simulink model "Mega_BalanceCode_r"  (R2023a)
settings: Solver=FixedStepDiscrete  StartTime=0.0  StopTime=inf  FixedStep=TS  RelTol=1e-3  EnableMultiTasking=on
values from neighbouring files (symbols this model uses):
  ES = -C2DEG*D2R    (= -0.00872664625997)    [NXT_Parameters.m]
  GS = GyroS*D2R    (= 0.000155832968928)    [NXT_Parameters.m]
  Ki = 1*[-Rw -Rw*0 1 1*0]    [NXT_Parameters.m]
  KLQRC = KLQR.*[-Rw -Rw 1 1]    [NXT_Parameters.m]
  TS = .005    (= 0.005)    [NXT_Parameters.m]
  tstart = TS*110    (= 0.55)    [NXT_Parameters.m]
  V2DCB = 1/DCB2V    (= 28.3333333333)    [NXT_Parameters.m]
undefined symbols (not defined in the file or in its folder): DiscIntNeverNeededParam
libraries: simulink x2, arduinolib x2
settings Model: FPTRunName=FPA_Reference  SimulationMode=external  ExtModeTrigDuration=2  Creator=Alec  LastModifiedBy=ASUS
settings SolverCC: AlgebraicLoopSolver=TrustRegion
settings DataIOCC: LimitDataPoints=on  SaveFormat=Array  ReturnWorkspaceOutputs=off
settings OptimizationCC: EnhancedBackFolding=on  PassReuseOutputArgsAs=Individual arguments  ExpressionDepthLimit=2147483647  ZeroExternalMemoryAtStartup=off  ZeroInternalMemoryAtStartup=off  MaxStackSize=64  OptimizeBlockOrder=speed  DifferentSizesBufferReuse=on  OptimizationCustomize=off  EfficientTunableParamExpr=on
settings DebuggingCC: UnderspecifiedInitializationDetection=Classic  MergeDetectMultiDrivingBlocksExec=none  ParameterTunabilityLossMsg=error  UnconnectedInputMsg=warning  UnconnectedOutputMsg=warning  UnconnectedLineMsg=warning  StateNameClashWarn=warning  SFUnexpectedBacktrackingDiag=warning  SFNoUnconditionalDefaultTransitionDiag=warning  SFExecutionAtInitializationDiag=none  ArithmeticOperatorsInVariantConditions=warning
settings HardwareCC: ProdBitPerInt=16  ProdBitPerPointer=16  ProdBitPerSizeT=16  ProdBitPerPtrDiffT=16  ProdLargestAtomicFloat=None  ProdWordSize=8  ProdHWDeviceType=Atmel->AVR
settings ModelReferenceCC: PropagateSignalLabelsOutOfModel=off
settings SFSimCC: SimUseLocalCustomCode=off  MATLABDynamicMemAlloc=off  CustomCodeUndefinedFunction=UseInterfaceOnly
settings RTWCC: Description=Embedded Coder  SystemTargetFile=ert.tlc  HardwareBoard=Arduino Mega 2560  TemplateMakefile=ert_default_tmf  RTWVerbose=off  RTWUseLocalCustomCode=off  Toolchain=Arduino AVR  BuildConfiguration=Faster Runs
settings CodeAppCC: ForceParamTrailComments=on  IgnoreCustomStorageClasses=off  OperatorAnnotations=on  SimulinkDataObjDesc=on  SFDataObjDesc=on  CustomSymbolStrType=$N$R$M  InsertBlockDesc=on  InternalIdentifier=Classic
settings ERTTargetCC: SupportContinuousTime=on  SupportVariableSizeSignals=on  ExtModeTransport=3  ExtModeStaticAlloc=on  ExtModeAutomaticAllocSize=off  ExtModeStaticAllocSize=2048  ExtModeMexFile=ext_xcp  ExtModeIntrfLevel=Level2 - Open
settings ConfigComp: CovMetricSettings=dw  CovSaveCumulativeToWorkspaceVar=on  CovSaveSingleToWorkspaceVar=on  CovExternalEMLEnable=off

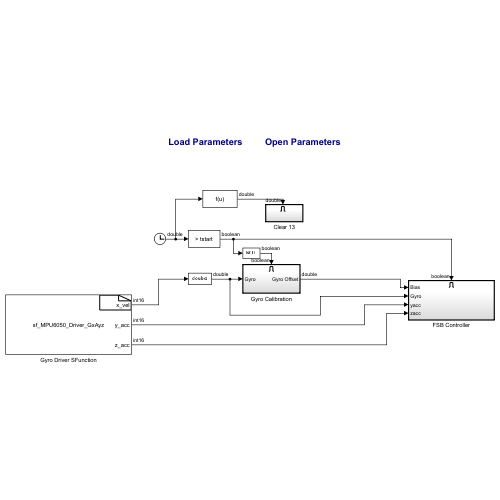
[thumbnail: Simulink's stored preview of the top-level diagram]
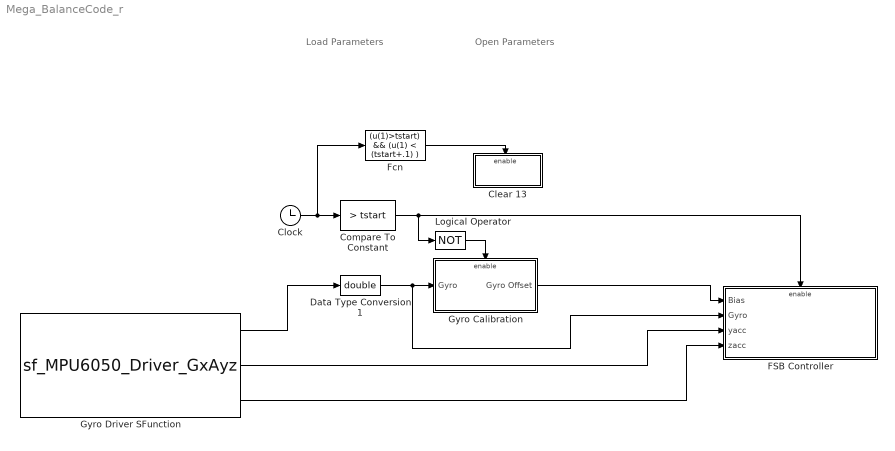
== system Mega_BalanceCode_r ==
  note: Load Parameters
  note: Open Parameters
  "Clear 13 " : Subsystem  TreatAsAtomicUnit=on
  Clock : Clock
  Compare To Constant : simulink/Logic and Bit Operations/Compare To Constant  relop=>  const=tstart  OutDataTypeStr=boolean
  Data Type Conversion1 : DataTypeConversion  OutDataTypeStr=double  SaturateOnIntegerOverflow=off  RndMeth=Floor
  FSB Controller : Subsystem
  Fcn : Fcn  Expr=(u(1)>tstart) && (u(1) < (tstart+.1) )
  Gyro Calibration : Subsystem  TreatAsAtomicUnit=on
  Gyro Driver SFunction : S-Function  InitFcn=try, set_param(gcb,'FunctionName','sf_MPU6050_Driver_GxAyz'), end  FunctionName=sf_MPU6050_Driver_GxAyz  SFunctionModules=sf_MPU6050_Driver_GxAyz_wrapper.cpp  SFunctionDeploymentMode=off  EnableBusSupport=off  mask(S-Function Builder){}
      mask help: Simulink:masks:SFunctionBuilder_MD
      mask init:
      | val = [[.9  0.75 0.75 1 1 .9 .9 1]',[1 1 0.75 0.75 .9 .9 1 .9]'];try , sys = get_param(gcb,'SfunBuilderFcnName');if isempty(sys), sys = get_param(gcb,'FunctionName'); end,catch, sys = get_param(gcb,'FunctionName'); end
      settings: CopyFcn=set_param(gcbh,'LinkStatus','none')  PreSaveFcn=try, set_param(gcb,'FunctionName','sf_MPU6050_Driver_GxAyz'), end  OpenFcn=sfunctionwizard(gcbh)
      mask Display:
      | plot(val(:,1),val(:,2))
      | disp(sys)
      | port_label('output',1,'x_vel')
      | port_label('output',2,'y_acc')
      | port_label('output',3,'z_acc')
  Logical Operator : Logic  Operator=NOT  AllPortsSameDT=off  OutDataTypeStr=boolean
  wires:
  Clock/1 -> Fcn/1, Compare To Constant/1
  Compare To Constant/1 -> Logical Operator/1, FSB Controller/Enable
  Gyro Calibration/1(Gyro Offset) -> FSB Controller/1(Bias)
  Gyro Driver SFunction/1 -> Data Type Conversion1/1
  Logical Operator/1 -> Gyro Calibration/Enable
  Data Type Conversion1/1 -> FSB Controller/2(Gyro), Gyro Calibration/1(Gyro)
  Fcn/1 -> "Clear 13 "/Enable
  Gyro Driver SFunction/2 -> FSB Controller/3("yacc ")
  Gyro Driver SFunction/3 -> FSB Controller/4("zacc ")

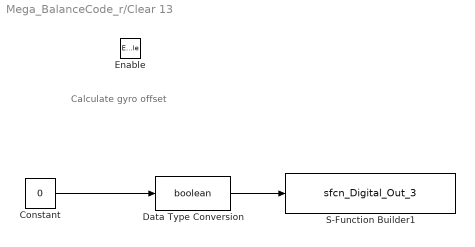
== system Mega_BalanceCode_r/Clear 13  ==
  note: Calculate gyro offset
  Enable : EnablePort
  Constant : Constant  Value=0
  Data Type Conversion : DataTypeConversion  OutDataTypeStr=boolean  SaturateOnIntegerOverflow=off  RndMeth=Floor
  S-Function Builder1 : S-Function  InitFcn=try, set_param(gcb,'FunctionName','sfcn_Digital_Out_3'), end  FunctionName=sfcn_Digital_Out_3  Parameters=uint8(13)  SFunctionModules=sfcn_Digital_Out_3_wrapper  SFunctionDeploymentMode=off  EnableBusSupport=off  mask(S-Function Builder){}
      mask init: same as Mega_BalanceCode_r/Gyro Driver SFunction
      settings: CopyFcn=set_param(gcbh,'LinkStatus','none')  PreSaveFcn=try, set_param(gcb,'FunctionName','sfcn_Digital_Out_3'), end  OpenFcn=sfunctionwizard(gcbh)
      mask Display: plot(val(:,1),val(:,2)),disp(sys), port_label('input',1,'in')
  wires:
  Constant/1 -> Data Type Conversion/1
  Data Type Conversion/1 -> S-Function Builder1/1

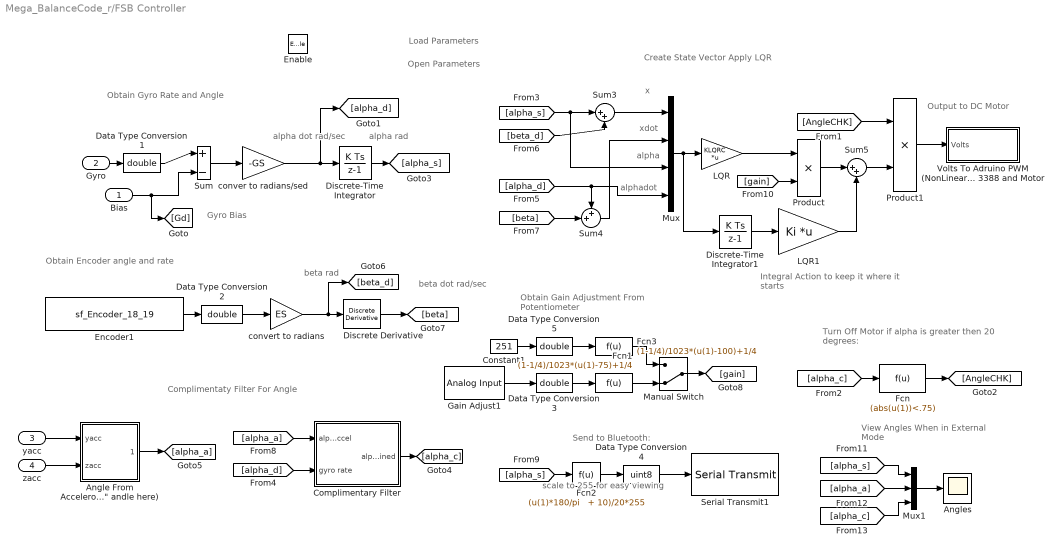
== system Mega_BalanceCode_r/FSB Controller ==
  note: scale to 255 for easy viewing
  note: Integral Action to keep
      |  it where it starts
  note: Gyro
      | Bias
  note: Turn Off Motor if alpha
      | is greater then 20 degrees:
  note: Output to DC Motor
  note: Create State Vector
      | Apply LQR
  note: Obtain Encoder angle
      | and rate
  note: Obtain Gyro Rate
      | and Angle
  note: xdot
  note: x
  note: beta
      | rad
  note: alpha dot
      | rad/sec
  note: alpha
      | rad
  note: beta dot
      | rad/sec
  note: alpha
  note: alphadot
  note: Load Parameters
  note: Open Parameters
  note: Complimentaty Filter
      | For Angle
  note: Obtain Gain Adjustment
      | From Potentiometer
  note: Send to Bluetooth:
  note: View Angles When in
      | External Mode
  Bias : Inport
  Gyro : Inport  Port=2
  "yacc " : Inport  Port=3
  "zacc " : Inport  Port=4
  Enable : EnablePort
  " Complimentary Filter" : Subsystem
  "Angle From Accelerometer (adjust \"zero\" andle here)" : Subsystem
  Angles : Scope
  Constant1 : Constant  Value=251
  Data Type Conversion{1..3,5} (4 alike) : DataTypeConversion  OutDataTypeStr=double  SaturateOnIntegerOverflow=off  RndMeth=Floor
  Data Type Conversion4 : DataTypeConversion  OutDataTypeStr=uint8  SaturateOnIntegerOverflow=off  RndMeth=Floor
  Discrete Derivative : simulink/Discrete/Discrete Derivative  gainval=1.0  ICPrevScaledInput=0.0  OutMin=[]  OutMax=[]  OutDataType=fixdt(1, 16)  OutScaling=2^-10  DoSatur=off
  Discrete-Time Integrator : DiscreteIntegrator  SampleTime=TS  ICPrevOutput=DiscIntNeverNeededParam  ICPrevScaledInput=DiscIntNeverNeededParam
  Discrete-Time Integrator1 : DiscreteIntegrator  SampleTime=TS  ICPrevOutput=DiscIntNeverNeededParam  ICPrevScaledInput=DiscIntNeverNeededParam
  Encoder1 : S-Function  InitFcn=try, set_param(gcb,'FunctionName','sf_Encoder_18_19'), end  FunctionName=sf_Encoder_18_19  Parameters=uint8(0),uint8(18),uint8(19)  SFunctionModules=sf_Encoder_18_19_wrapper  SFunctionDeploymentMode=off  EnableBusSupport=off  mask(S-Function Builder){}
      mask init: same as Mega_BalanceCode_r/Gyro Driver SFunction
      settings: CopyFcn=set_param(gcbh,'LinkStatus','none')  PreSaveFcn=try, set_param(gcb,'FunctionName','sf_Encoder_18_19'), end  OpenFcn=sfunctionwizard(gcbh)
      mask Display: plot(val(:,1),val(:,2)),disp(sys), port_label('output',1,'pos')
  Fcn : Fcn  Expr=(abs(u(1))<.75)
  Fcn1 : Fcn  Expr=(1-1/4)/1023*(u(1)-75)+1/4
  Fcn2 : Fcn  Expr="(u(1)*180/pi   + 10)/20*255"
  Fcn3 : Fcn  Expr=(1-1/4)/1023*(u(1)-100)+1/4
  Gain Adjust1 : arduinolib/Analog Input  pinNumber=13  ReadResultsOnly=off  ConversionTriggerSource=Software  ExternalTriggerType=uint32( 0 )  OutputDataType=uint16  EnableConversionCompleteNotify=off  EnableOuputStatus=off  SampleTime=-1  blockPlatform=arduino
  LQR : Gain  Gain=KLQRC  Multiplication=Matrix(K*u)
  LQR1 : Gain  Gain=Ki  Multiplication=Matrix(K*u)
  Manual Switch : ManualSwitch  CurrentSetting=0
  Mux : Mux
  Mux1 : Mux  Inputs=3
  Product : Product  RndMeth=Zero
  Product1 : Product  RndMeth=Zero
  Serial Transmit1 : arduinolib/Serial Transmit  portNumber=3  sendmode=write  sendformat=Decimal  floatprecision=2  blockPlatform=arduino
  Sum : Sum  Inputs=|+-
  Sum3 : Sum  Inputs=|++
  Sum4 : Sum  Inputs=++|
  Sum5 : Sum  Inputs=|++
  Volts To Adruino PWM (NonLinear LOW) 3388 and Motor : Subsystem
  conver to radians/sed : Gain  Gain=-GS
  convert to radians : Gain  Gain=ES  OutDataTypeStr=double
  wires:
  Sum3/1 -> Mux/1
  Data Type Conversion2/1 -> convert to radians/1
  Bias/1 -> [Gd], Sum/2
  Sum/1 -> conver to radians/sed/1
  Fcn/1 -> [AngleCHK]
  Encoder1/1 -> Data Type Conversion2/1
  Mux/1 -> Discrete-Time Integrator1/1, LQR/1
  Data Type Conversion1/1 -> Sum/1
  [alpha_c] -> Fcn/1
  conver to radians/sed/1 -> Discrete-Time Integrator/1, [alpha_d]
  Sum4/1 -> Mux/2
  Discrete-Time Integrator/1 -> [alpha_s]
  Fcn2/1 -> Data Type Conversion4/1
  Data Type Conversion4/1 -> Serial Transmit1/1
  [alpha_s] -> Sum3/1, Mux/3
  Discrete-Time Integrator1/1 -> LQR1/1
  Product/1 -> Sum5/1
  LQR/1 -> Product/1
  Sum5/1 -> Product1/2
  [AngleCHK] -> Product1/1
  LQR1/1 -> Sum5/2
  Gyro/1 -> Data Type Conversion1/1
  [alpha_a] -> " Complimentary Filter"/1(alpha accel)
  [alpha_d] -> " Complimentary Filter"/2(gyro rate)
  [alpha_d] -> Mux/4, Sum4/1
  convert to radians/1 -> Discrete Derivative/1, [beta_d]
  Discrete Derivative/1 -> [beta]
  [beta] -> Sum4/2
  [beta_d] -> Sum3/2
  [alpha_s] -> Fcn2/1
  Data Type Conversion3/1 -> Fcn1/1
  Gain Adjust1/1 -> Data Type Conversion3/1
  Fcn1/1 -> Manual Switch/2
  Constant1/1 -> Data Type Conversion5/1
  Data Type Conversion5/1 -> Fcn3/1
  Fcn3/1 -> Manual Switch/1
  Manual Switch/1 -> [gain]
  [gain] -> Product/2
  Product1/1 -> Volts To Adruino PWM (NonLinear LOW) 3388 and Motor/1(Volts)
  [alpha_s] -> Mux1/1
  [alpha_a] -> Mux1/2
  [alpha_c] -> Mux1/3
  Mux1/1 -> Angles/1
  "yacc "/1 -> "Angle From Accelerometer (adjust \"zero\" andle here)"/1(yacc)
  "zacc "/1 -> "Angle From Accelerometer (adjust \"zero\" andle here)"/2(zacc)
  "Angle From Accelerometer (adjust \"zero\" andle here)"/1(angle rad) -> [alpha_a]
  " Complimentary Filter"/1(alpha combined) -> [alpha_c]

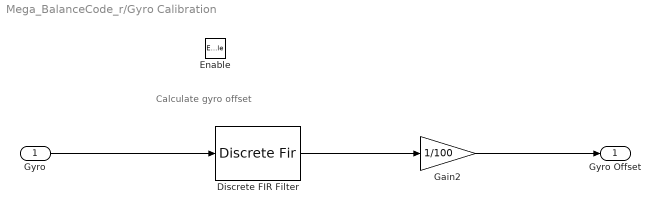
== system Mega_BalanceCode_r/Gyro Calibration ==
  note: Calculate gyro offset
  Gyro : Inport
  Enable : EnablePort
  Discrete FIR Filter : DiscreteFir  Coefficients=ones(1,100)
  Gain2 : Gain  Gain=1/100  OutDataTypeStr=Inherit: Same as input  ParamDataTypeStr=Inherit: Same as input
  Gyro Offset : Outport
  wires:
  Gyro/1 -> Discrete FIR Filter/1
  Discrete FIR Filter/1 -> Gain2/1
  Gain2/1 -> Gyro Offset/1

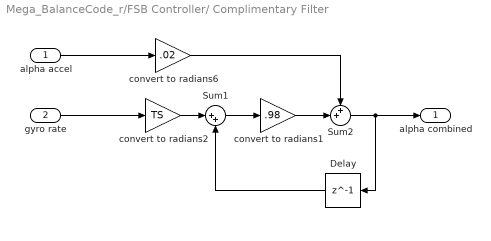
== system Mega_BalanceCode_r/FSB Controller/ Complimentary Filter ==
  alpha accel : Inport
  gyro rate : Inport  Port=2
  Delay : Delay  DelayLength=1  SampleTime=TS
  Sum1 : Sum  Inputs=|++
  Sum2 : Sum  Inputs=++|
  convert to radians1 : Gain  Gain=.98  OutDataTypeStr=double
  convert to radians2 : Gain  Gain=TS  OutDataTypeStr=double
  convert to radians6 : Gain  Gain=.02  OutDataTypeStr=double
  alpha combined : Outport
  wires:
  gyro rate/1 -> convert to radians2/1
  Sum1/1 -> convert to radians1/1
  convert to radians6/1 -> Sum2/1
  alpha accel/1 -> convert to radians6/1
  convert to radians1/1 -> Sum2/2
  Delay/1 -> Sum1/2
  convert to radians2/1 -> Sum1/1
  Sum2/1 -> Delay/1, alpha combined/1

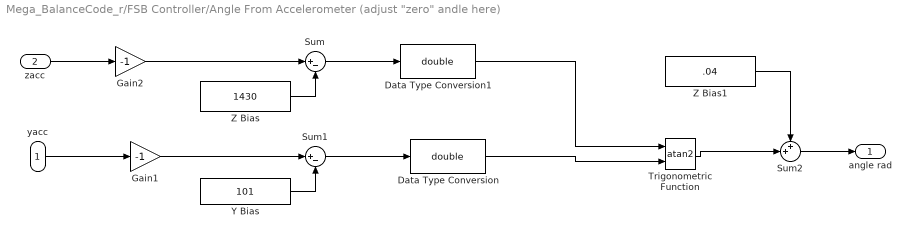
== system Mega_BalanceCode_r/FSB Controller/Angle From Accelerometer (adjust "zero" andle here) ==
  yacc : Inport
  zacc : Inport  Port=2
  Data Type Conversion : DataTypeConversion  OutDataTypeStr=double  SaturateOnIntegerOverflow=off  RndMeth=Floor
  Data Type Conversion1 : DataTypeConversion  OutDataTypeStr=double  SaturateOnIntegerOverflow=off  RndMeth=Floor
  Gain1 : Gain  Gain=-1
  Gain2 : Gain  Gain=-1
  Sum : Sum  Inputs=|+-
  Sum1 : Sum  Inputs=|+-
  Sum2 : Sum  Inputs=++|
  Trigonometric Function : Trigonometry  Operator=atan2
  Y Bias : Constant  Value=101
  Z Bias : Constant  Value=1430
  Z Bias1 : Constant  Value=.04
  angle rad : Outport
  wires:
  Sum1/1 -> Data Type Conversion/1
  Gain2/1 -> Sum/1
  Sum/1 -> Data Type Conversion1/1
  Z Bias/1 -> Sum/2
  Gain1/1 -> Sum1/1
  Y Bias/1 -> Sum1/2
  zacc/1 -> Gain2/1
  yacc/1 -> Gain1/1
  Trigonometric Function/1 -> Sum2/2
  Sum2/1 -> angle rad/1
  Z Bias1/1 -> Sum2/1
  Data Type Conversion1/1 -> Trigonometric Function/1
  Data Type Conversion/1 -> Trigonometric Function/2

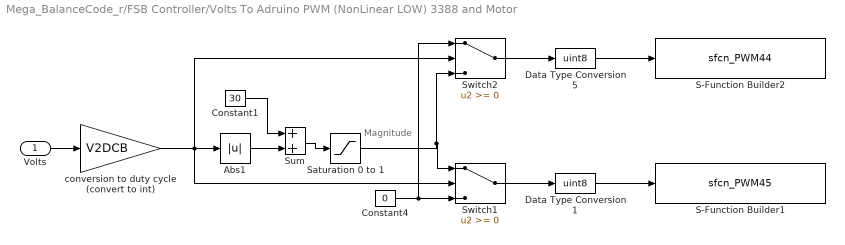
== system Mega_BalanceCode_r/FSB Controller/Volts To Adruino PWM (NonLinear LOW) 3388 and Motor ==
  note: Magnitude
  Volts : Inport
  Abs1 : Abs  SaturateOnIntegerOverflow=off
  Constant1 : Constant  Value=30
  Constant4 : Constant  Value=0
  Data Type Conversion1 : DataTypeConversion  OutDataTypeStr=uint8  SaturateOnIntegerOverflow=off  RndMeth=Floor
  Data Type Conversion5 : DataTypeConversion  OutDataTypeStr=uint8  SaturateOnIntegerOverflow=off  RndMeth=Floor
  S-Function Builder1 : S-Function  InitFcn=try, set_param(gcb,'FunctionName','sfcn_PWM45'), end  FunctionName=sfcn_PWM45  Parameters=uint8(45)  SFunctionModules=sfcn_PWM45_wrapper  SFunctionDeploymentMode=off  EnableBusSupport=off  mask(S-Function Builder){}
      mask init: same as Mega_BalanceCode_r/Gyro Driver SFunction
      settings: CopyFcn=set_param(gcbh,'LinkStatus','none')  PreSaveFcn=try, set_param(gcb,'FunctionName','sfcn_PWM45'), end  OpenFcn=sfunctionwizard(gcbh)
      mask Display: plot(val(:,1),val(:,2)),disp(sys), port_label('input',1,'in')
  S-Function Builder2 : S-Function  InitFcn=try, set_param(gcb,'FunctionName','sfcn_PWM44'), end  FunctionName=sfcn_PWM44  Parameters=uint8(44)  SFunctionModules=sfcn_PWM44_wrapper  SFunctionDeploymentMode=off  EnableBusSupport=off  mask(S-Function Builder){}
      mask init: same as Mega_BalanceCode_r/Gyro Driver SFunction
      settings: CopyFcn=set_param(gcbh,'LinkStatus','none')  PreSaveFcn=try, set_param(gcb,'FunctionName','sfcn_PWM44'), end  OpenFcn=sfunctionwizard(gcbh)
      mask Display: plot(val(:,1),val(:,2)),disp(sys), port_label('input',1,'in')
  Saturation 0 to 1 : Saturate  UpperLimit=255  LowerLimit=0
  Sum : Sum
  Switch1 : Switch  SaturateOnIntegerOverflow=off  InputSameDT=off
  Switch2 : Switch  SaturateOnIntegerOverflow=off  InputSameDT=off
  conversion to duty cycle (convert to int) : Gain  Gain=V2DCB  OutDataTypeStr=int16
  wires:
  Volts/1 -> conversion to duty cycle (convert to int)/1
  conversion to duty cycle (convert to int)/1 -> Switch1/2, Abs1/1, Switch2/2
  Constant4/1 -> Switch2/1, Switch1/3
  Saturation 0 to 1/1 -> Switch2/3, Switch1/1
  Switch2/1 -> Data Type Conversion5/1
  Switch1/1 -> Data Type Conversion1/1
  Data Type Conversion5/1 -> S-Function Builder2/1
  Data Type Conversion1/1 -> S-Function Builder1/1
  Abs1/1 -> Sum/2
  Sum/1 -> Saturation 0 to 1/1
  Constant1/1 -> Sum/1
